simulink model "dc_motor_scratch"  (R2025a)
settings: Solver=ode23t  StartTime=0.0  StopTime=10.0  RelTol=1e-3  AbsTol=1e-3  EnableMultiTasking=on
libraries: fl_lib x12, nesl_utility x2
CloseFcn:
  | try,close(h1_dc_motor_scratch),end
  | clear h1_dc_motor_scratch
  | try,close(h2_dc_motor_scratch),end
  | clear h2_dc_motor_scratch
  | 
  | clear simlog_dc_motor_scratch
Description:
  | Copyright 2016-2025 The MathWorks, Inc.
settings Model: Creator=smiller  LastModifiedBy=smiller
settings SolverCC: AutoScaleAbsTol=off  AlgebraicLoopSolver=TrustRegion
settings DataIOCC: MaxDataPoints=10000  ReturnWorkspaceOutputs=off  SignalLoggingName=logsout_dc_motor_scratch
settings OptimizationCC: ReuseModelBlockBuffer=off  LifeSpan=inf
settings DebuggingCC: UnconnectedInputMsg=warning  UnconnectedOutputMsg=warning  UnconnectedLineMsg=warning  PregeneratedLibrarySubsystemCodeDiagnostic=none  SFUnexpectedBacktrackingDiag=warning  SFNoUnconditionalDefaultTransitionDiag=warning  SFExecutionAtInitializationDiag=none  ArithmeticOperatorsInVariantConditions=warning
settings ModelReferenceCC: EnableRefExpFcnMdlSchedulingChecks=on
settings SFSimCC: SimUseLocalCustomCode=off  CustomCodeUndefinedFunction=UseInterfaceOnly
settings RTWCC: RTWUseLocalCustomCode=off  GPUComputeCapability=3.5  DLArmComputeVersion=19.05
settings CodeAppCC: StateflowObjectComments=on
settings GRTTargetCC: TargetLangStandard=C89/C90 (ANSI)
settings ConfigComp: CovMetricSettings=dw  CovSaveCumulativeToWorkspaceVar=on  CovSaveSingleToWorkspaceVar=on  CovExternalEMLEnable=off
settings SimscapeCC: SimscapeNormalizeSystem=off  SimscapeNominalValues="[{\"value\":\"10\",\"unit\":\"V\"},{\"value\":\"1\",\"unit\":\"A\"},{\"value\":\"10\",\"unit\":\"N*m\"},{\"value\":\"10\",\"unit\":\"bar\"},{\"value\":\"100\",\"unit\":\"kJ/kg\"},{\"value\":\"1\",\"unit\":\"kW\"},{\"value\":\"300\",\"unit\":\"K\"},{\"value\":\"100\",\"unit\":\"cm^3/s\"},{\"value\":\"1\",\"unit\":\"kN\"},{\"value\":\"1\",\"unit\":\"g/cm^3\"},{\"value\":\"1\",\"unit\":\"l\"},{\"value\":\"1\",\"unit\":\"cm^2\"},{\"value\":\"60\",\"unit\":\"Hz\"}]"  SimscapeLogType=all  SimscapeLogSimulationStatistics=on  SimscapeLogName=simlog_dc_motor_scratch  SimscapeLogDataHistory=10000.0

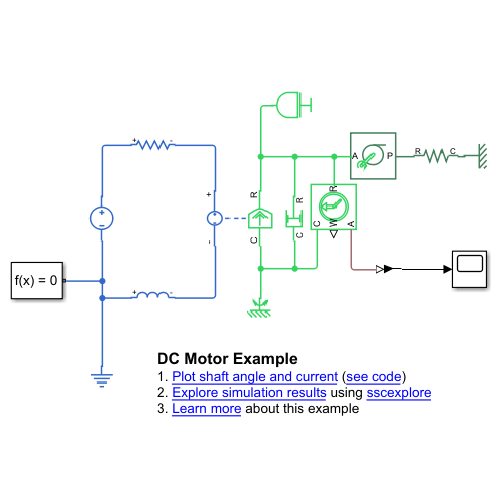
[thumbnail: Simulink's stored preview of the top-level diagram]
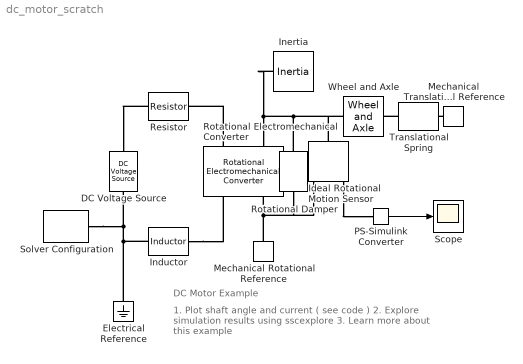
== system dc_motor_scratch ==
  note: DC Motor Example
  note: 1. Plot shaft angle and current ( see code )
      | 2. Explore simulation results using sscexplore
      | 3. Learn more about this example
  DC Voltage Source : fl_lib/Electrical/Electrical Sources/DC Voltage Source  v0=5 V
  Electrical Reference : fl_lib/Electrical/Electrical Elements/Electrical Reference
  Ideal Rotational Motion Sensor : fl_lib/Mechanical/Mechanical Sensors/Ideal Rotational Motion Sensor  reference=foundation.enum.MeasurementReference.difference  acceleration_port=false  velocity_port=true  position_port=true  wrap_angle=simscape.enum.onoff.off  offset=0 rad
  Inductor : fl_lib/Electrical/Electrical Elements/Inductor  l=1e-6 H  r=0 Ohm  g=1e-9 1/Ohm  i_specify=off  i_priority=None  i=0 A  i_nominal_specify=off  i_nominal_value=1  i_nominal_unit=A  v_specify=off  v_priority=None  v=0 V  v_nominal_specify=off  v_nominal_value=1  v_nominal_unit=V  i_L_specify=off  i_L_priority=High  i_L=0 A  i_L_nominal_specify=off  i_L_nominal_value=1  i_L_nominal_unit=A
  Inertia : fl_lib/Mechanical/Rotational Elements/Inertia  inertia=0.01 kg*m^2  num_ports=foundation.enum.numPorts2.one  w_specify=off  w_priority=High  w=0 rad/s  w_nominal_specify=off  w_nominal_value=1  w_nominal_unit=rad/s  t_specify=off  t_priority=None  t=0 N*m  t_nominal_specify=off  t_nominal_value=1  t_nominal_unit=N*m
  Mechanical Rotational Reference : fl_lib/Mechanical/Rotational Elements/Mechanical Rotational Reference
  Mechanical Translational Reference : fl_lib/Mechanical/Translational Elements/Mechanical Translational Reference
  PS-Simulink Converter : nesl_utility/PS-Simulink Converter  PhysicalDomain=network_engine_domain  SubClassName=ps_output  LeftPortType=input  RightPortType=output  PseudoPeriodic=off  Frequencies=[]  VectorFormat=1-D array  Unit=deg  AffineConversion=off
  Resistor : fl_lib/Electrical/Electrical Elements/Resistor  R=1 Ohm  i_specify=off  i_priority=None  i=0 A  i_nominal_specify=off  i_nominal_value=1  i_nominal_unit=A  v_specify=off  v_priority=None  v=0 V  v_nominal_specify=off  v_nominal_value=1  v_nominal_unit=V
  Rotational Electromechanical Converter : fl_lib/Electrical/Electrical Elements/Rotational Electromechanical Converter  K=0.1 V/(rad/s)  i_specify=off  i_priority=None  i=0 A  i_nominal_specify=off  i_nominal_value=1  i_nominal_unit=A  v_specify=off  v_priority=None  v=0 V  v_nominal_specify=off  v_nominal_value=1  v_nominal_unit=V  t_specify=off  t_priority=None  t=0 N*m  t_nominal_specify=off  t_nominal_value=1  t_nominal_unit=N*m  w_specify=off  w_priority=None  w=0 rad/s  w_nominal_specify=off  w_nominal_value=1  w_nominal_unit=rad/s
  Rotational Damper : fl_lib/Mechanical/Rotational Elements/Rotational Damper  D=0.001 N*m/(rad/s)  w_specify=off  w_priority=None  w=0 rad/s  w_nominal_specify=off  w_nominal_value=1  w_nominal_unit=rad/s  t_specify=off  t_priority=None  t=0 N*m  t_nominal_specify=off  t_nominal_value=1  t_nominal_unit=N*m
  Scope : Scope
      settings: ActiveDisplayYMinimum=-5.32013  ActiveDisplayYMaximum=47.88119
  Solver Configuration : nesl_utility/Solver Configuration  PhysicalDomain=network_engine_domain  SubClassName=solver  LeftPortType=input  RightPortType=generic  Tones=[]  Harmonics=[]  SimulateNoise=off  Profile=off  UseLocalSampling=off  EnableSwitchedLinearOptims=on  FrequencyDomain=off  UseCCode=off  RelTol=0.001  AbsTol=1e-06  MinStep=1e-09  ToWorkspace=off  RevertToSquareIcSolve=off  NumHomotopyIterations=100  PhasorMode=off  PhasorModeNumHarmonics=1  ConsistencySolver=NEWTON_FTOL  IndexReductionMethod=DerivativeReplacement  DoDC=off  ResidualTolerance=1e-09  ConsistencyTolSource=GLOBAL  ConsistencyAbsTol=0.001  ConsistencyRelTol=0.001  ConsistencyTolFactor=0.001  UseLocalSolver=off  LocalSolverChoice=NE_BACKWARD_EULER_ADVANCER  ResolveIndetEquations=on  FunctionEvalNumThread=1  LocalSolverSampleTime=0.001  DoFixedCost=off  MaxNonlinIter=3  MaxModeIter=2  ComputeImpulses=off  ImpulseIterations=2  LinearAlgebra=Sparse  LinearAlgebraNumThread=0  EquationFormulation=NE_TIME_EF  DelaysMemoryBudget=1024  AutomaticFiltering=on  FilteringTimeConstant=0.001  PartitionStorageMethod=AS_NEEDED  PartitionMemoryBudget=1024  PartitionMethod=FAST  MultibodyUseLocalSolver=off  MultibodyLocalSolverChoice=ODE1  MultibodyLocalSolverSampleTime=0.001
  Translational Spring : fl_lib/Mechanical/Translational Elements/Translational Spring  spr_rate=500 N/m  v_specify=off  v_priority=None  v=0 m/s  v_nominal_specify=off  v_nominal_value=1  v_nominal_unit=m/s  f_specify=off  f_priority=None  f=0 N  f_nominal_specify=off  f_nominal_value=1  f_nominal_unit=N  x_specify=off  x_priority=High  x=0 m  x_nominal_specify=off  x_nominal_value=1  x_nominal_unit=m
  Wheel and Axle : fl_lib/Mechanical/Mechanisms/Wheel and Axle  R=0.05 m  or=1  t_specify=off  t_priority=None  t=0 N*m  t_nominal_specify=off  t_nominal_value=1  t_nominal_unit=N*m  f_specify=off  f_priority=None  f=0 N  f_nominal_specify=off  f_nominal_value=1  f_nominal_unit=N
  wires:
  PS-Simulink Converter/1 -> Scope/1
  connections:
  Resistor/LConn1 -- DC Voltage Source/LConn1
  Rotational Electromechanical Converter/LConn1 -- Resistor/RConn1
  Inductor/LConn1 -- Electrical Reference/LConn1 -- Solver Configuration/RConn1 -- DC Voltage Source/RConn1
  Inductor/RConn1 -- Rotational Electromechanical Converter/RConn1
  Mechanical Rotational Reference/LConn1 -- Ideal Rotational Motion Sensor/RConn1 -- Rotational Damper/RConn1 -- Rotational Electromechanical Converter/RConn2
  Inertia/LConn1 -- Wheel and Axle/LConn1 -- Ideal Rotational Motion Sensor/LConn1 -- Rotational Damper/LConn1 -- Rotational Electromechanical Converter/LConn2
  Translational Spring/LConn1 -- Wheel and Axle/RConn1
  Mechanical Translational Reference/LConn1 -- Translational Spring/RConn1
  Ideal Rotational Motion Sensor/RConn3 -- PS-Simulink Converter/LConn1
